simulink model "moteur_inertie"  (R2026a)
settings: Solver=FixedStepAuto  StopTime=5  FixedStep=1/1000
values from neighbouring files (symbols this model uses):
  coef_sec = 0.1    [parametres_moteur.m]
  coef_visq = 0.2    [parametres_moteur.m]
  J = 5e-2    (= 0.05)    [parametres_moteur.m]
  Ke = 0.8    [parametres_moteur.m]
  Kt = 0.8    [parametres_moteur.m]
  L = 2e-3    (= 0.002)    [parametres_moteur.m]
  R = 2    [parametres_moteur.m]
  U = 28    [parametres_moteur.m]
settings Model: Creator=lulu1  LastModifiedBy=lulu1

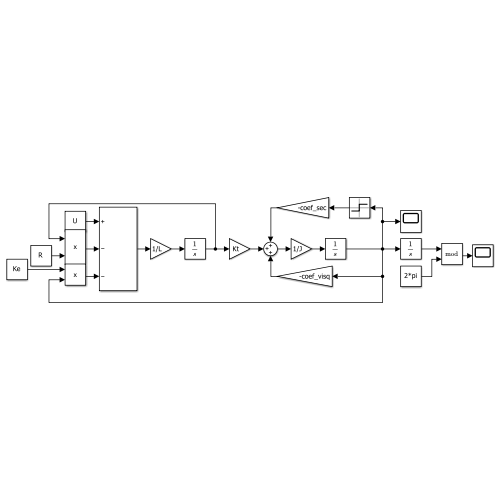
[thumbnail: Simulink's stored preview of the top-level diagram]
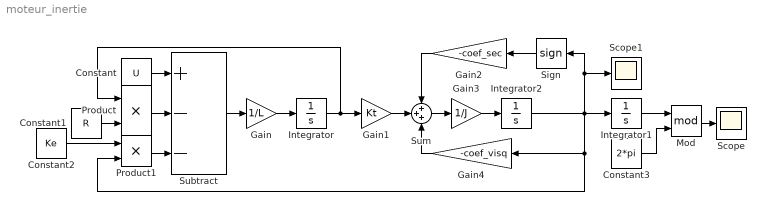
== system moteur_inertie ==
  Constant : Constant  Value=U
  Constant1 : Constant  Value=R
  Constant2 : Constant  Value=Ke
  Constant3 : Constant  Value=2*pi
  Gain : Gain  Gain=1/L
  Gain1 : Gain  Gain=Kt
  Gain2 : Gain  Gain=-coef_sec
  Gain3 : Gain  Gain=1/J
  Gain4 : Gain  Gain=-coef_visq
  Integrator : Integrator
  Integrator1 : Integrator
  Integrator2 : Integrator
  Mod : Math  Operator=mod
  Product : Product
  Product1 : Product
  Scope : Scope
      settings: ActiveDisplayYMinimum=-1.2565659211070082  ActiveDisplayYMaximum=6.5969710858117931
  Scope1 : Scope
      settings: ActiveDisplayYMinimum=-2.6682692307692095  ActiveDisplayYMaximum=24.014423076922888
  Sign : Signum
  Subtract : Sum  Inputs=+--
  Sum : Sum  Inputs=+++
  wires:
  Product/1 -> Subtract/2
  Constant1/1 -> Product/2
  Gain/1 -> Integrator/1
  Subtract/1 -> Gain/1
  Constant/1 -> Subtract/1
  Integrator/1 -> Gain1/1, Product/1
  Integrator2/1 -> Product1/2, Gain4/1, Sign/1, Scope1/1, Integrator1/1
  Constant2/1 -> Product1/1
  Product1/1 -> Subtract/3
  Integrator1/1 -> Mod/1
  Constant3/1 -> Mod/2
  Mod/1 -> Scope/1
  Gain3/1 -> Integrator2/1
  Sum/1 -> Gain3/1
  Gain1/1 -> Sum/2
  Sign/1 -> Gain2/1
  Gain2/1 -> Sum/1
  Gain4/1 -> Sum/3
